simulink model "voltage_measure"  (R2022b)
settings: Solver=ode1be  StartTime=0.0  StopTime=200e-3  FixedStep=1e-6  RelTol=1e-3
libraries: fl_lib x68, nesl_utility x7
settings Model: Creator=ltnbda  LastModifiedBy=ltnbda

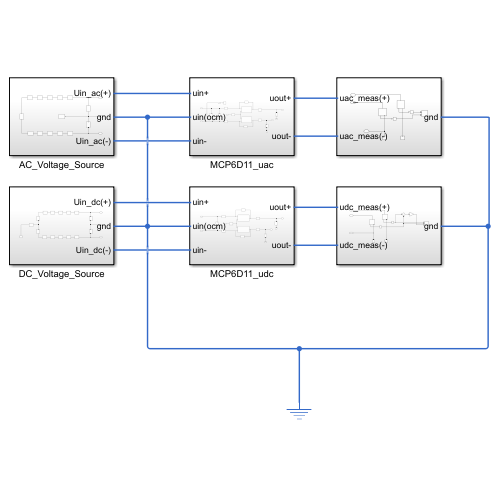
[thumbnail: Simulink's stored preview of the top-level diagram]
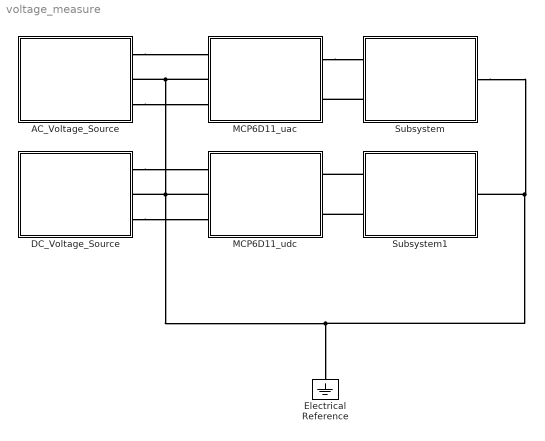
== system voltage_measure ==
  AC_Voltage_Source : Subsystem
  DC_Voltage_Source : Subsystem
  Electrical Reference : fl_lib/Electrical/Electrical Elements/Electrical Reference
  MCP6D11_uac : Subsystem
  MCP6D11_udc : Subsystem
  Subsystem : Subsystem
  Subsystem1 : Subsystem
  connections:
  MCP6D11_uac/RConn1 -- Subsystem/LConn1
  Subsystem/LConn2 -- MCP6D11_uac/RConn2
  Subsystem1/LConn1 -- MCP6D11_udc/RConn1
  Subsystem1/LConn2 -- MCP6D11_udc/RConn2
  AC_Voltage_Source/RConn1 -- MCP6D11_uac/LConn1
  AC_Voltage_Source/RConn3 -- MCP6D11_uac/LConn3
  DC_Voltage_Source/RConn1 -- MCP6D11_udc/LConn1
  DC_Voltage_Source/RConn3 -- MCP6D11_udc/LConn3
  Subsystem/RConn1 -- Electrical Reference/LConn1 -- AC_Voltage_Source/RConn2 -- MCP6D11_uac/LConn2 -- MCP6D11_udc/LConn2 -- DC_Voltage_Source/RConn2 -- Subsystem1/RConn1

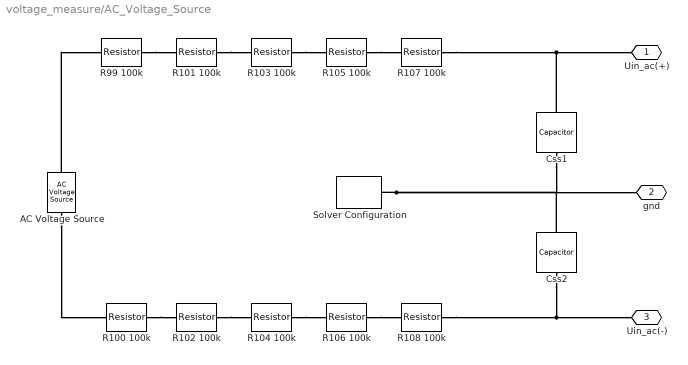
== system voltage_measure/AC_Voltage_Source ==
  AC Voltage Source : fl_lib/Electrical/Electrical Sources/AC Voltage Source  amp=1350 V  shift=0 deg  frequency=50 Hz  omega=0 rad/s
  Css1 : fl_lib/Electrical/Electrical Elements/Capacitor  c=12e-12 F  r=1e-6 Ohm  g=0 1/Ohm  i_specify=off  i_priority=None  i=0 A  i_nominal_specify=off  i_nominal_unit=A  i_nominal_value=1  v_specify=off  v_priority=None  v=0 V  v_nominal_specify=off  v_nominal_unit=V  v_nominal_value=1  vc_specify=off  vc_priority=High  vc=0 V  vc_nominal_specify=off  vc_nominal_unit=V  vc_nominal_value=1
  Css2 : fl_lib/Electrical/Electrical Elements/Capacitor  c=12e-12 F  r=1e-6 Ohm  g=0 1/Ohm  i_specify=off  i_priority=None  i=0 A  i_nominal_specify=off  i_nominal_unit=A  i_nominal_value=1  v_specify=off  v_priority=None  v=0 V  v_nominal_specify=off  v_nominal_unit=V  v_nominal_value=1  vc_specify=off  vc_priority=High  vc=0 V  vc_nominal_specify=off  vc_nominal_unit=V  vc_nominal_value=1
  R100 100k : fl_lib/Electrical/Electrical Elements/Resistor  R=127e3/2 Ohm  i_specify=off  i_priority=None  i=0 A  i_nominal_specify=off  i_nominal_unit=A  i_nominal_value=1  v_specify=off  v_priority=None  v=0 V  v_nominal_specify=off  v_nominal_unit=V  v_nominal_value=1
  R101 100k : fl_lib/Electrical/Electrical Elements/Resistor  R=127e3/2 Ohm  i_specify=off  i_priority=None  i=0 A  i_nominal_specify=off  i_nominal_unit=A  i_nominal_value=1  v_specify=off  v_priority=None  v=0 V  v_nominal_specify=off  v_nominal_unit=V  v_nominal_value=1
  R102 100k : fl_lib/Electrical/Electrical Elements/Resistor  R=127e3/2 Ohm  i_specify=off  i_priority=None  i=0 A  i_nominal_specify=off  i_nominal_unit=A  i_nominal_value=1  v_specify=off  v_priority=None  v=0 V  v_nominal_specify=off  v_nominal_unit=V  v_nominal_value=1
  R103 100k : fl_lib/Electrical/Electrical Elements/Resistor  R=127e3/2 Ohm  i_specify=off  i_priority=None  i=0 A  i_nominal_specify=off  i_nominal_unit=A  i_nominal_value=1  v_specify=off  v_priority=None  v=0 V  v_nominal_specify=off  v_nominal_unit=V  v_nominal_value=1
  R104 100k : fl_lib/Electrical/Electrical Elements/Resistor  R=127e3/2 Ohm  i_specify=off  i_priority=None  i=0 A  i_nominal_specify=off  i_nominal_unit=A  i_nominal_value=1  v_specify=off  v_priority=None  v=0 V  v_nominal_specify=off  v_nominal_unit=V  v_nominal_value=1
  R105 100k : fl_lib/Electrical/Electrical Elements/Resistor  R=127e3/2 Ohm  i_specify=off  i_priority=None  i=0 A  i_nominal_specify=off  i_nominal_unit=A  i_nominal_value=1  v_specify=off  v_priority=None  v=0 V  v_nominal_specify=off  v_nominal_unit=V  v_nominal_value=1
  R106 100k : fl_lib/Electrical/Electrical Elements/Resistor  R=127e3/2 Ohm  i_specify=off  i_priority=None  i=0 A  i_nominal_specify=off  i_nominal_unit=A  i_nominal_value=1  v_specify=off  v_priority=None  v=0 V  v_nominal_specify=off  v_nominal_unit=V  v_nominal_value=1
  R107 100k : fl_lib/Electrical/Electrical Elements/Resistor  R=127e3/2 Ohm  i_specify=off  i_priority=None  i=0 A  i_nominal_specify=off  i_nominal_unit=A  i_nominal_value=1  v_specify=off  v_priority=None  v=0 V  v_nominal_specify=off  v_nominal_unit=V  v_nominal_value=1
  R108 100k : fl_lib/Electrical/Electrical Elements/Resistor  R=127e3/2 Ohm  i_specify=off  i_priority=None  i=0 A  i_nominal_specify=off  i_nominal_unit=A  i_nominal_value=1  v_specify=off  v_priority=None  v=0 V  v_nominal_specify=off  v_nominal_unit=V  v_nominal_value=1
  R99 100k : fl_lib/Electrical/Electrical Elements/Resistor  R=127e3/2 Ohm  i_specify=off  i_priority=None  i=0 A  i_nominal_specify=off  i_nominal_unit=A  i_nominal_value=1  v_specify=off  v_priority=None  v=0 V  v_nominal_specify=off  v_nominal_unit=V  v_nominal_value=1
  Solver Configuration : nesl_utility/Solver Configuration  PhysicalDomain=network_engine_domain  SubClassName=solver  LeftPortType=input  RightPortType=generic  Tones=[]  Harmonics=[]  SimulateNoise=off  Profile=off  UseLocalSampling=off  EnableSwitchedLinearOptims=on  FrequencyDomain=off  UseCCode=off  RelTol=0.001  AbsTol=0.001  MinStep=1e-09  ToWorkspace=off  RevertToSquareIcSolve=off  NumHomotopyIterations=100  PhasorMode=off  PhasorModeNumHarmonics=1  ConsistencySolver=NEWTON_XTOL_AFTER_FTOL  IndexReductionMethod=DerivativeReplacement  DoDC=off  ResidualTolerance=1e-09  ConsistencyTolSource=GLOBAL  ConsistencyAbsTol=0.001  ConsistencyRelTol=0.001  ConsistencyTolFactor=0.001  UseLocalSolver=on  LocalSolverChoice=NE_BACKWARD_EULER_ADVANCER  ResolveIndetEquations=on  FunctionEvalNumThread=1  LocalSolverSampleTime=1e-6  DoFixedCost=on  MaxNonlinIter=3  MaxModeIter=2  ComputeImpulses=off  ImpulseIterations=2  LinearAlgebra=auto  LinearAlgebraNumThread=0  EquationFormulation=NE_TIME_EF  DelaysMemoryBudget=1024  AutomaticFiltering=on  FilteringTimeConstant=0.001  PartitionStorageMethod=AS_NEEDED  PartitionMemoryBudget=1024  PartitionMethod=ROBUST
  Uin_ac(+) : PMIOPort  Side=Right
  gnd : PMIOPort  Port=2  Side=Right
  Uin_ac(-) : PMIOPort  Port=3  Side=Right
  connections:
  AC Voltage Source/RConn1 -- R100 100k/LConn1
  R99 100k/RConn1 -- R101 100k/LConn1
  AC Voltage Source/LConn1 -- R99 100k/LConn1
  R105 100k/RConn1 -- R107 100k/LConn1
  R101 100k/RConn1 -- R103 100k/LConn1
  R103 100k/RConn1 -- R105 100k/LConn1
  R107 100k/RConn1 -- Css1/LConn1 -- Uin_ac(+)/RConn1
  R100 100k/RConn1 -- R102 100k/LConn1
  R106 100k/RConn1 -- R108 100k/LConn1
  R102 100k/RConn1 -- R104 100k/LConn1
  R104 100k/RConn1 -- R106 100k/LConn1
  R108 100k/RConn1 -- Css2/RConn1 -- Uin_ac(-)/RConn1
  Solver Configuration/RConn1 -- Css2/LConn1 -- Css1/RConn1 -- gnd/RConn1

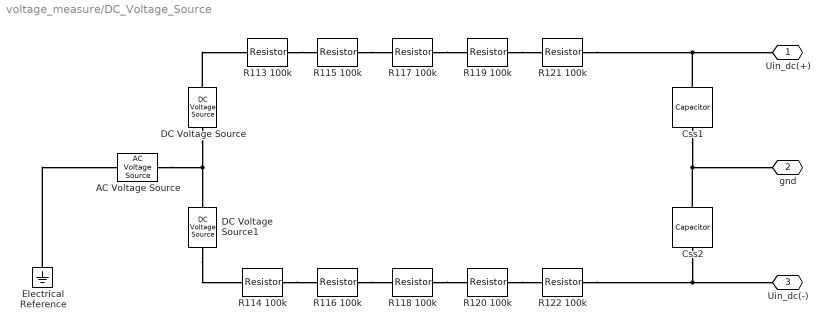
== system voltage_measure/DC_Voltage_Source ==
  AC Voltage Source : fl_lib/Electrical/Electrical Sources/AC Voltage Source  amp=500 V  shift=0 deg  frequency=4000 Hz  omega=0 rad/s
  Css1 : fl_lib/Electrical/Electrical Elements/Capacitor  c=12e-12 F  r=1e-6 Ohm  g=0 1/Ohm  i_specify=off  i_priority=None  i=0 A  i_nominal_specify=off  i_nominal_unit=A  i_nominal_value=1  v_specify=off  v_priority=None  v=0 V  v_nominal_specify=off  v_nominal_unit=V  v_nominal_value=1  vc_specify=off  vc_priority=High  vc=0 V  vc_nominal_specify=off  vc_nominal_unit=V  vc_nominal_value=1
  Css2 : fl_lib/Electrical/Electrical Elements/Capacitor  c=12e-12 F  r=1e-6 Ohm  g=0 1/Ohm  i_specify=off  i_priority=None  i=0 A  i_nominal_specify=off  i_nominal_unit=A  i_nominal_value=1  v_specify=off  v_priority=None  v=0 V  v_nominal_specify=off  v_nominal_unit=V  v_nominal_value=1  vc_specify=off  vc_priority=High  vc=0 V  vc_nominal_specify=off  vc_nominal_unit=V  vc_nominal_value=1
  DC Voltage Source : fl_lib/Electrical/Electrical Sources/DC Voltage Source  v0=1070/2 V
  DC Voltage Source1 : fl_lib/Electrical/Electrical Sources/DC Voltage Source  v0=1070/2 V
  Electrical Reference : fl_lib/Electrical/Electrical Elements/Electrical Reference
  R113 100k : fl_lib/Electrical/Electrical Elements/Resistor  R=127e3/2 Ohm  i_specify=off  i_priority=None  i=0 A  i_nominal_specify=off  i_nominal_unit=A  i_nominal_value=1  v_specify=off  v_priority=None  v=0 V  v_nominal_specify=off  v_nominal_unit=V  v_nominal_value=1
  R114 100k : fl_lib/Electrical/Electrical Elements/Resistor  R=127e3/2 Ohm  i_specify=off  i_priority=None  i=0 A  i_nominal_specify=off  i_nominal_unit=A  i_nominal_value=1  v_specify=off  v_priority=None  v=0 V  v_nominal_specify=off  v_nominal_unit=V  v_nominal_value=1
  R115 100k : fl_lib/Electrical/Electrical Elements/Resistor  R=127e3/2 Ohm  i_specify=off  i_priority=None  i=0 A  i_nominal_specify=off  i_nominal_unit=A  i_nominal_value=1  v_specify=off  v_priority=None  v=0 V  v_nominal_specify=off  v_nominal_unit=V  v_nominal_value=1
  R116 100k : fl_lib/Electrical/Electrical Elements/Resistor  R=127e3/2 Ohm  i_specify=off  i_priority=None  i=0 A  i_nominal_specify=off  i_nominal_unit=A  i_nominal_value=1  v_specify=off  v_priority=None  v=0 V  v_nominal_specify=off  v_nominal_unit=V  v_nominal_value=1
  R117 100k : fl_lib/Electrical/Electrical Elements/Resistor  R=127e3/2 Ohm  i_specify=off  i_priority=None  i=0 A  i_nominal_specify=off  i_nominal_unit=A  i_nominal_value=1  v_specify=off  v_priority=None  v=0 V  v_nominal_specify=off  v_nominal_unit=V  v_nominal_value=1
  R118 100k : fl_lib/Electrical/Electrical Elements/Resistor  R=127e3/2 Ohm  i_specify=off  i_priority=None  i=0 A  i_nominal_specify=off  i_nominal_unit=A  i_nominal_value=1  v_specify=off  v_priority=None  v=0 V  v_nominal_specify=off  v_nominal_unit=V  v_nominal_value=1
  R119 100k : fl_lib/Electrical/Electrical Elements/Resistor  R=127e3/2 Ohm  i_specify=off  i_priority=None  i=0 A  i_nominal_specify=off  i_nominal_unit=A  i_nominal_value=1  v_specify=off  v_priority=None  v=0 V  v_nominal_specify=off  v_nominal_unit=V  v_nominal_value=1
  R120 100k : fl_lib/Electrical/Electrical Elements/Resistor  R=127e3/2 Ohm  i_specify=off  i_priority=None  i=0 A  i_nominal_specify=off  i_nominal_unit=A  i_nominal_value=1  v_specify=off  v_priority=None  v=0 V  v_nominal_specify=off  v_nominal_unit=V  v_nominal_value=1
  R121 100k : fl_lib/Electrical/Electrical Elements/Resistor  R=127e3/2 Ohm  i_specify=off  i_priority=None  i=0 A  i_nominal_specify=off  i_nominal_unit=A  i_nominal_value=1  v_specify=off  v_priority=None  v=0 V  v_nominal_specify=off  v_nominal_unit=V  v_nominal_value=1
  R122 100k : fl_lib/Electrical/Electrical Elements/Resistor  R=127e3/2 Ohm  i_specify=off  i_priority=None  i=0 A  i_nominal_specify=off  i_nominal_unit=A  i_nominal_value=1  v_specify=off  v_priority=None  v=0 V  v_nominal_specify=off  v_nominal_unit=V  v_nominal_value=1
  Uin_dc(+) : PMIOPort  Side=Right
  gnd : PMIOPort  Port=2  Side=Right
  Uin_dc(-) : PMIOPort  Port=3  Side=Right
  connections:
  R122 100k/RConn1 -- Css2/RConn1 -- Uin_dc(-)/RConn1
  R118 100k/RConn1 -- R120 100k/LConn1
  R116 100k/RConn1 -- R118 100k/LConn1
  R120 100k/RConn1 -- R122 100k/LConn1
  R114 100k/RConn1 -- R116 100k/LConn1
  R121 100k/RConn1 -- Css1/LConn1 -- Uin_dc(+)/RConn1
  R117 100k/RConn1 -- R119 100k/LConn1
  R115 100k/RConn1 -- R117 100k/LConn1
  R119 100k/RConn1 -- R121 100k/LConn1
  DC Voltage Source/LConn1 -- R113 100k/LConn1
  R113 100k/RConn1 -- R115 100k/LConn1
  DC Voltage Source/RConn1 -- DC Voltage Source1/LConn1 -- AC Voltage Source/LConn1
  Css1/RConn1 -- gnd/RConn1 -- Css2/LConn1
  DC Voltage Source1/RConn1 -- R114 100k/LConn1
  Electrical Reference/LConn1 -- AC Voltage Source/RConn1

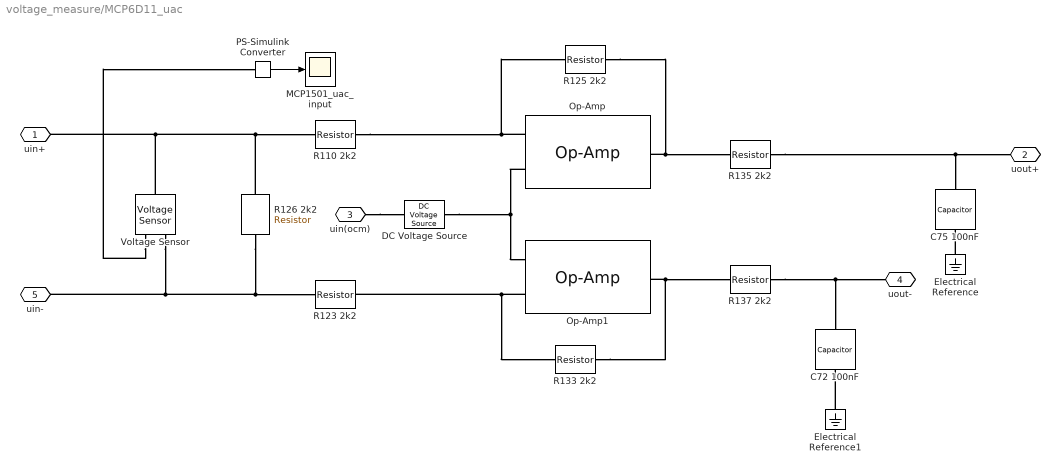
== system voltage_measure/MCP6D11_uac ==
  C72 100nF : fl_lib/Electrical/Electrical Elements/Capacitor  c=100e-9 F  r=1e-6 Ohm  g=0 1/Ohm  i_specify=off  i_priority=None  i=0 A  i_nominal_specify=off  i_nominal_unit=A  i_nominal_value=1  v_specify=off  v_priority=None  v=0 V  v_nominal_specify=off  v_nominal_unit=V  v_nominal_value=1  vc_specify=off  vc_priority=High  vc=0 V  vc_nominal_specify=off  vc_nominal_unit=V  vc_nominal_value=1
  C75 100nF : fl_lib/Electrical/Electrical Elements/Capacitor  c=100e-9 F  r=1e-6 Ohm  g=0 1/Ohm  i_specify=off  i_priority=None  i=0 A  i_nominal_specify=off  i_nominal_unit=A  i_nominal_value=1  v_specify=off  v_priority=None  v=0 V  v_nominal_specify=off  v_nominal_unit=V  v_nominal_value=1  vc_specify=off  vc_priority=High  vc=0 V  vc_nominal_specify=off  vc_nominal_unit=V  vc_nominal_value=1
  DC Voltage Source : fl_lib/Electrical/Electrical Sources/DC Voltage Source  v0=1.5 V
  Electrical Reference : fl_lib/Electrical/Electrical Elements/Electrical Reference
  Electrical Reference1 : fl_lib/Electrical/Electrical Elements/Electrical Reference
  MCP1501_uac_input : Scope
  Op-Amp : fl_lib/Electrical/Electrical Elements/Op-Amp  outI_specify=off  outI_priority=None  outI=0 A  outI_nominal_specify=off  outI_nominal_unit=A  outI_nominal_value=1
  Op-Amp1 : fl_lib/Electrical/Electrical Elements/Op-Amp  outI_specify=off  outI_priority=None  outI=0 A  outI_nominal_specify=off  outI_nominal_unit=A  outI_nominal_value=1
  PS-Simulink Converter : nesl_utility/PS-Simulink Converter  PhysicalDomain=network_engine_domain  SubClassName=ps_output  LeftPortType=input  RightPortType=output  PseudoPeriodic=off  Frequencies=[]  VectorFormat=1-D array  Unit=V  AffineConversion=off
  R110 2k2 : fl_lib/Electrical/Electrical Elements/Resistor  R=2.2e3 Ohm  i_specify=off  i_priority=None  i=0 A  i_nominal_specify=off  i_nominal_unit=A  i_nominal_value=1  v_specify=off  v_priority=None  v=0 V  v_nominal_specify=off  v_nominal_unit=V  v_nominal_value=1
  R123 2k2 : fl_lib/Electrical/Electrical Elements/Resistor  R=2.2e3 Ohm  i_specify=off  i_priority=None  i=0 A  i_nominal_specify=off  i_nominal_unit=A  i_nominal_value=1  v_specify=off  v_priority=None  v=0 V  v_nominal_specify=off  v_nominal_unit=V  v_nominal_value=1
  R125 2k2 : fl_lib/Electrical/Electrical Elements/Resistor  R=2.2e3 Ohm  i_specify=off  i_priority=None  i=0 A  i_nominal_specify=off  i_nominal_unit=A  i_nominal_value=1  v_specify=off  v_priority=None  v=0 V  v_nominal_specify=off  v_nominal_unit=V  v_nominal_value=1
  R126 2k2 : fl_lib/Electrical/Electrical Elements/Resistor  R=2.2e3 Ohm  i_specify=off  i_priority=None  i=0 A  i_nominal_specify=off  i_nominal_unit=A  i_nominal_value=1  v_specify=off  v_priority=None  v=0 V  v_nominal_specify=off  v_nominal_unit=V  v_nominal_value=1
  R133 2k2 : fl_lib/Electrical/Electrical Elements/Resistor  R=2.2e3 Ohm  i_specify=off  i_priority=None  i=0 A  i_nominal_specify=off  i_nominal_unit=A  i_nominal_value=1  v_specify=off  v_priority=None  v=0 V  v_nominal_specify=off  v_nominal_unit=V  v_nominal_value=1
  R135 2k2 : fl_lib/Electrical/Electrical Elements/Resistor  R=2.2e3 Ohm  i_specify=off  i_priority=None  i=0 A  i_nominal_specify=off  i_nominal_unit=A  i_nominal_value=1  v_specify=off  v_priority=None  v=0 V  v_nominal_specify=off  v_nominal_unit=V  v_nominal_value=1
  R137 2k2 : fl_lib/Electrical/Electrical Elements/Resistor  R=2.2e3 Ohm  i_specify=off  i_priority=None  i=0 A  i_nominal_specify=off  i_nominal_unit=A  i_nominal_value=1  v_specify=off  v_priority=None  v=0 V  v_nominal_specify=off  v_nominal_unit=V  v_nominal_value=1
  Voltage Sensor : fl_lib/Electrical/Electrical Sensors/Voltage Sensor
  uin+ : PMIOPort  Side=Left
  uout+ : PMIOPort  Port=2  Side=Right
  uin(ocm) : PMIOPort  Port=3  Side=Left
  uout- : PMIOPort  Port=4  Side=Right
  uin- : PMIOPort  Port=5  Side=Left
  wires:
  PS-Simulink Converter/1 -> MCP1501_uac_input/1
  connections:
  Op-Amp1/LConn2 -- R133 2k2/LConn1 -- R123 2k2/RConn1
  R126 2k2/LConn1 -- Voltage Sensor/LConn1 -- uin+/RConn1 -- R110 2k2/LConn1
  Op-Amp/LConn2 -- R125 2k2/LConn1 -- R110 2k2/RConn1
  Op-Amp/LConn1 -- DC Voltage Source/LConn1 -- Op-Amp1/LConn1
  R125 2k2/RConn1 -- R135 2k2/LConn1 -- Op-Amp/RConn1
  R137 2k2/RConn1 -- uout-/RConn1 -- C72 100nF/LConn1
  R126 2k2/RConn1 -- Voltage Sensor/RConn2 -- uin-/RConn1 -- R123 2k2/LConn1
  Electrical Reference1/LConn1 -- C72 100nF/RConn1
  Electrical Reference/LConn1 -- C75 100nF/RConn1
  R135 2k2/RConn1 -- uout+/RConn1 -- C75 100nF/LConn1
  R133 2k2/RConn1 -- R137 2k2/LConn1 -- Op-Amp1/RConn1
  Voltage Sensor/RConn1 -- PS-Simulink Converter/LConn1
  uin(ocm)/RConn1 -- DC Voltage Source/RConn1

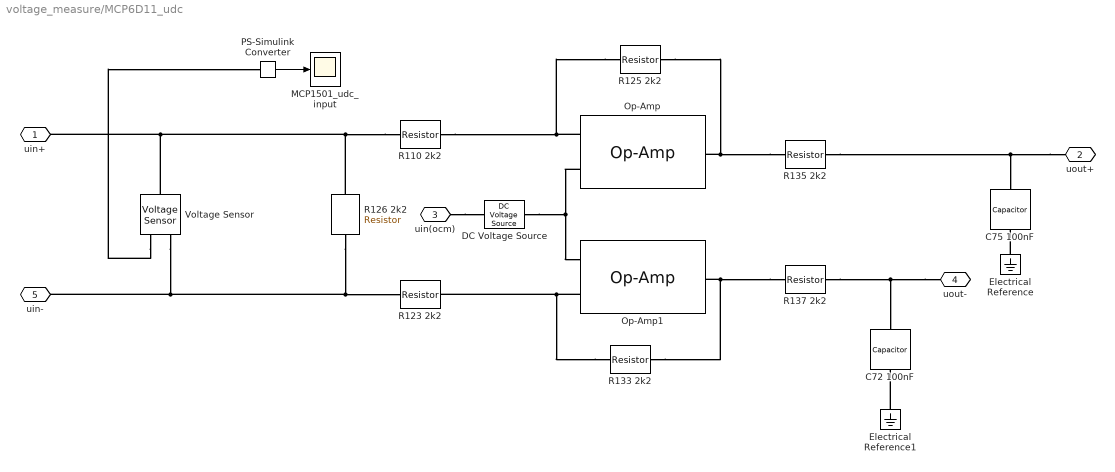
== system voltage_measure/MCP6D11_udc ==
  C72 100nF : fl_lib/Electrical/Electrical Elements/Capacitor  c=100e-9 F  r=1e-6 Ohm  g=0 1/Ohm  i_specify=off  i_priority=None  i=0 A  i_nominal_specify=off  i_nominal_unit=A  i_nominal_value=1  v_specify=off  v_priority=None  v=0 V  v_nominal_specify=off  v_nominal_unit=V  v_nominal_value=1  vc_specify=off  vc_priority=High  vc=0 V  vc_nominal_specify=off  vc_nominal_unit=V  vc_nominal_value=1
  C75 100nF : fl_lib/Electrical/Electrical Elements/Capacitor  c=100e-9 F  r=1e-6 Ohm  g=0 1/Ohm  i_specify=off  i_priority=None  i=0 A  i_nominal_specify=off  i_nominal_unit=A  i_nominal_value=1  v_specify=off  v_priority=None  v=0 V  v_nominal_specify=off  v_nominal_unit=V  v_nominal_value=1  vc_specify=off  vc_priority=High  vc=0 V  vc_nominal_specify=off  vc_nominal_unit=V  vc_nominal_value=1
  DC Voltage Source : fl_lib/Electrical/Electrical Sources/DC Voltage Source  v0=1.5 V
  Electrical Reference : fl_lib/Electrical/Electrical Elements/Electrical Reference
  Electrical Reference1 : fl_lib/Electrical/Electrical Elements/Electrical Reference
  MCP1501_udc_input : Scope
  Op-Amp : fl_lib/Electrical/Electrical Elements/Op-Amp  outI_specify=off  outI_priority=None  outI=0 A  outI_nominal_specify=off  outI_nominal_unit=A  outI_nominal_value=1
  Op-Amp1 : fl_lib/Electrical/Electrical Elements/Op-Amp  outI_specify=off  outI_priority=None  outI=0 A  outI_nominal_specify=off  outI_nominal_unit=A  outI_nominal_value=1
  PS-Simulink Converter : nesl_utility/PS-Simulink Converter  PhysicalDomain=network_engine_domain  SubClassName=ps_output  LeftPortType=input  RightPortType=output  PseudoPeriodic=off  Frequencies=[]  VectorFormat=1-D array  Unit=V  AffineConversion=off
  R110 2k2 : fl_lib/Electrical/Electrical Elements/Resistor  R=2.2e3 Ohm  i_specify=off  i_priority=None  i=0 A  i_nominal_specify=off  i_nominal_unit=A  i_nominal_value=1  v_specify=off  v_priority=None  v=0 V  v_nominal_specify=off  v_nominal_unit=V  v_nominal_value=1
  R123 2k2 : fl_lib/Electrical/Electrical Elements/Resistor  R=2.2e3 Ohm  i_specify=off  i_priority=None  i=0 A  i_nominal_specify=off  i_nominal_unit=A  i_nominal_value=1  v_specify=off  v_priority=None  v=0 V  v_nominal_specify=off  v_nominal_unit=V  v_nominal_value=1
  R125 2k2 : fl_lib/Electrical/Electrical Elements/Resistor  R=2.2e3 Ohm  i_specify=off  i_priority=None  i=0 A  i_nominal_specify=off  i_nominal_unit=A  i_nominal_value=1  v_specify=off  v_priority=None  v=0 V  v_nominal_specify=off  v_nominal_unit=V  v_nominal_value=1
  R126 2k2 : fl_lib/Electrical/Electrical Elements/Resistor  R=2.2e3 Ohm  i_specify=off  i_priority=None  i=0 A  i_nominal_specify=off  i_nominal_unit=A  i_nominal_value=1  v_specify=off  v_priority=None  v=0 V  v_nominal_specify=off  v_nominal_unit=V  v_nominal_value=1
  R133 2k2 : fl_lib/Electrical/Electrical Elements/Resistor  R=2.2e3 Ohm  i_specify=off  i_priority=None  i=0 A  i_nominal_specify=off  i_nominal_unit=A  i_nominal_value=1  v_specify=off  v_priority=None  v=0 V  v_nominal_specify=off  v_nominal_unit=V  v_nominal_value=1
  R135 2k2 : fl_lib/Electrical/Electrical Elements/Resistor  R=2.2e3 Ohm  i_specify=off  i_priority=None  i=0 A  i_nominal_specify=off  i_nominal_unit=A  i_nominal_value=1  v_specify=off  v_priority=None  v=0 V  v_nominal_specify=off  v_nominal_unit=V  v_nominal_value=1
  R137 2k2 : fl_lib/Electrical/Electrical Elements/Resistor  R=2.2e3 Ohm  i_specify=off  i_priority=None  i=0 A  i_nominal_specify=off  i_nominal_unit=A  i_nominal_value=1  v_specify=off  v_priority=None  v=0 V  v_nominal_specify=off  v_nominal_unit=V  v_nominal_value=1
  Voltage Sensor : fl_lib/Electrical/Electrical Sensors/Voltage Sensor
  uin+ : PMIOPort  Side=Left
  uout+ : PMIOPort  Port=2  Side=Right
  uin(ocm) : PMIOPort  Port=3  Side=Left
  uout- : PMIOPort  Port=4  Side=Right
  uin- : PMIOPort  Port=5  Side=Left
  wires:
  PS-Simulink Converter/1 -> MCP1501_udc_input/1
  connections:
  R137 2k2/LConn1 -- Op-Amp1/RConn1 -- R133 2k2/RConn1
  uout+/RConn1 -- R135 2k2/RConn1 -- C75 100nF/LConn1
  Electrical Reference/LConn1 -- C75 100nF/RConn1
  Electrical Reference1/LConn1 -- C72 100nF/RConn1
  R126 2k2/RConn1 -- Voltage Sensor/RConn2 -- uin-/RConn1 -- R123 2k2/LConn1
  uout-/RConn1 -- R137 2k2/RConn1 -- C72 100nF/LConn1
  R135 2k2/LConn1 -- Op-Amp/RConn1 -- R125 2k2/RConn1
  Op-Amp/LConn1 -- DC Voltage Source/LConn1 -- Op-Amp1/LConn1
  R125 2k2/LConn1 -- Op-Amp/LConn2 -- R110 2k2/RConn1
  R110 2k2/LConn1 -- uin+/RConn1 -- Voltage Sensor/LConn1 -- R126 2k2/LConn1
  R133 2k2/LConn1 -- R123 2k2/RConn1 -- Op-Amp1/LConn2
  uin(ocm)/RConn1 -- DC Voltage Source/RConn1
  Voltage Sensor/RConn1 -- PS-Simulink Converter/LConn1

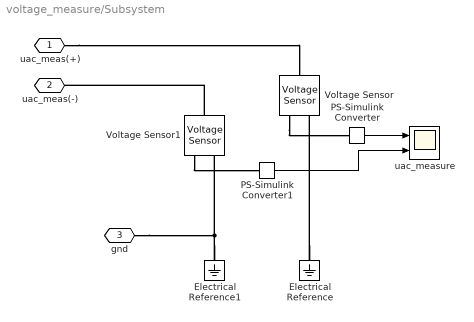
== system voltage_measure/Subsystem ==
  Electrical Reference : fl_lib/Electrical/Electrical Elements/Electrical Reference
  Electrical Reference1 : fl_lib/Electrical/Electrical Elements/Electrical Reference
  PS-Simulink Converter : nesl_utility/PS-Simulink Converter  PhysicalDomain=network_engine_domain  SubClassName=ps_output  LeftPortType=input  RightPortType=output  PseudoPeriodic=off  Frequencies=[]  VectorFormat=1-D array  Unit=V  AffineConversion=off
  PS-Simulink Converter1 : nesl_utility/PS-Simulink Converter  PhysicalDomain=network_engine_domain  SubClassName=ps_output  LeftPortType=input  RightPortType=output  PseudoPeriodic=off  Frequencies=[]  VectorFormat=1-D array  Unit=V  AffineConversion=off
  Voltage Sensor : fl_lib/Electrical/Electrical Sensors/Voltage Sensor
  Voltage Sensor1 : fl_lib/Electrical/Electrical Sensors/Voltage Sensor
  uac_measure : Scope  NumInputPorts=2
  uac_meas(+) : PMIOPort  Side=Left
  uac_meas(-) : PMIOPort  Port=2  Side=Left
  gnd : PMIOPort  Port=3  Side=Right
  wires:
  PS-Simulink Converter/1 -> uac_measure/1
  PS-Simulink Converter1/1 -> uac_measure/2
  connections:
  Voltage Sensor1/RConn1 -- PS-Simulink Converter1/LConn1
  Electrical Reference/LConn1 -- Voltage Sensor/RConn2
  uac_meas(+)/RConn1 -- Voltage Sensor/LConn1
  Voltage Sensor/RConn1 -- PS-Simulink Converter/LConn1
  Electrical Reference1/LConn1 -- gnd/RConn1 -- Voltage Sensor1/RConn2
  Voltage Sensor1/LConn1 -- uac_meas(-)/RConn1

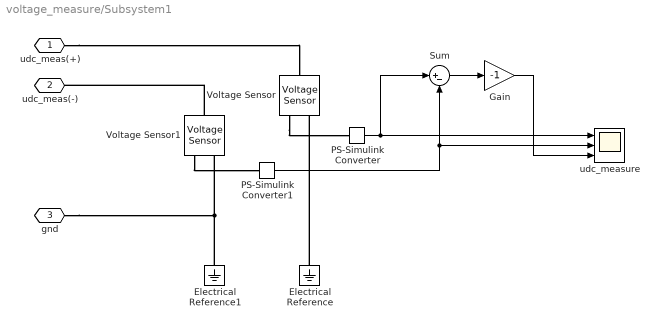
== system voltage_measure/Subsystem1 ==
  Electrical Reference : fl_lib/Electrical/Electrical Elements/Electrical Reference
  Electrical Reference1 : fl_lib/Electrical/Electrical Elements/Electrical Reference
  Gain : Gain  Gain=-1
  PS-Simulink Converter : nesl_utility/PS-Simulink Converter  PhysicalDomain=network_engine_domain  SubClassName=ps_output  LeftPortType=input  RightPortType=output  PseudoPeriodic=off  Frequencies=[]  VectorFormat=1-D array  Unit=V  AffineConversion=off
  PS-Simulink Converter1 : nesl_utility/PS-Simulink Converter  PhysicalDomain=network_engine_domain  SubClassName=ps_output  LeftPortType=input  RightPortType=output  PseudoPeriodic=off  Frequencies=[]  VectorFormat=1-D array  Unit=V  AffineConversion=off
  Sum : Sum  Inputs=|+-
  Voltage Sensor : fl_lib/Electrical/Electrical Sensors/Voltage Sensor
  Voltage Sensor1 : fl_lib/Electrical/Electrical Sensors/Voltage Sensor
  udc_measure : Scope  NumInputPorts=3
  udc_meas(+) : PMIOPort  Side=Left
  udc_meas(-) : PMIOPort  Port=2  Side=Left
  gnd : PMIOPort  Port=3  Side=Right
  wires:
  PS-Simulink Converter1/1 -> Sum/2, udc_measure/2
  PS-Simulink Converter/1 -> Sum/1, udc_measure/1
  Sum/1 -> Gain/1
  Gain/1 -> udc_measure/3
  connections:
  Voltage Sensor1/LConn1 -- udc_meas(-)/RConn1
  Electrical Reference1/LConn1 -- gnd/RConn1 -- Voltage Sensor1/RConn2
  Voltage Sensor/RConn1 -- PS-Simulink Converter/LConn1
  udc_meas(+)/RConn1 -- Voltage Sensor/LConn1
  Electrical Reference/LConn1 -- Voltage Sensor/RConn2
  Voltage Sensor1/RConn1 -- PS-Simulink Converter1/LConn1
